simulink model "redundant_leg_final"  (R2024a)
settings: Solver=ode23tb  StartTime=0.0  StopTime=1  RelTol=1e-3
libraries: spsMosfetLib x6, spsIdealSwitchLib x4, spsCurrentMeasurementLib x3, spsDCVoltageSourceLib x1, spsSeriesRLCBranchLib x1, spsTriangleGeneratorLib x1, spsVoltageMeasurementLib x1, sps_lib x1
settings Model: Creator=student  LastModifiedBy=Rupa
settings SolverCC: ZeroCrossControl=DisableAll
settings RTWCC: GPUComputeCapability=3.5

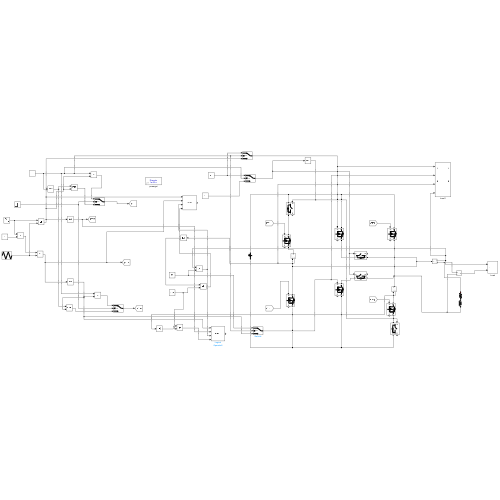
[thumbnail: Simulink's stored preview of the top-level diagram]
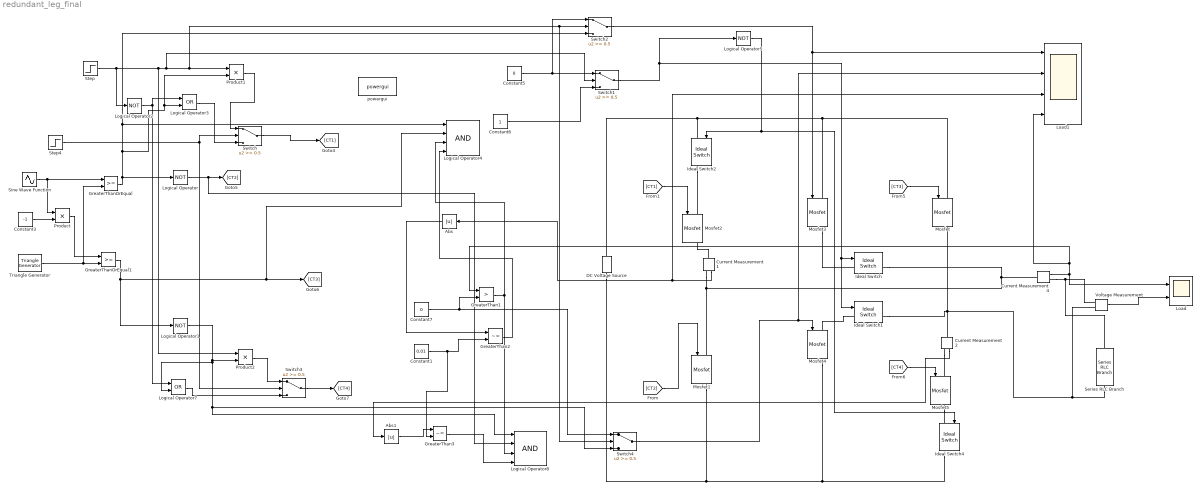
== system redundant_leg_final ==
  Abs : Abs  SaturateOnIntegerOverflow=off
  Abs1 : Abs  SaturateOnIntegerOverflow=off
  Constant1 : Constant  Value=0.01
  Constant3 : Constant  Value=-1
  Constant5 : Constant  Value=0
  Constant6 : Constant
  Constant7 : Constant  Value=0
  Current Measurement1 : spsCurrentMeasurementLib/Current Measurement  PhasorSimulation=off  OutputType=Complex  PSBequivalent=0
  Current Measurement2 : spsCurrentMeasurementLib/Current Measurement  PhasorSimulation=off  OutputType=Complex  PSBequivalent=0
  Current Measurement4 : spsCurrentMeasurementLib/Current Measurement  PhasorSimulation=off  OutputType=Complex  PSBequivalent=0
  DC Voltage Source : spsDCVoltageSourceLib/DC Voltage Source  Amplitude=200  Measurements=None
  GreaterThan1 : RelationalOperator  Operator=>  OutDataTypeStr=boolean  RndMeth=Simplest  InputSameDT=off
  GreaterThan2 : RelationalOperator  Operator=~=  OutDataTypeStr=boolean  RndMeth=Simplest  InputSameDT=off
  GreaterThan3 : RelationalOperator  Operator=~=  OutDataTypeStr=boolean  RndMeth=Simplest  InputSameDT=off
  GreaterThanOrEqual : RelationalOperator  OutDataTypeStr=boolean  RndMeth=Simplest  InputSameDT=off
  GreaterThanOrEqual1 : RelationalOperator  OutDataTypeStr=boolean  RndMeth=Simplest  InputSameDT=off
  Ideal Switch{,1..2,4} (4 alike) : spsIdealSwitchLib/Ideal Switch  Ron=0.001  Lon=0  IC=0  Rs=1e5  Cs=inf  Measurements=on
  Load : Scope  NumInputPorts=2
  Load1 : Scope  NumInputPorts=4
  Logical Operator{,1..2,5} (4 alike) : Logic  Operator=NOT  AllPortsSameDT=off  OutDataTypeStr=boolean
  Logical Operator3 : Logic  Operator=OR  AllPortsSameDT=off  OutDataTypeStr=boolean
  Logical Operator4 : Logic  Inputs=4  AllPortsSameDT=off  OutDataTypeStr=boolean
  Logical Operator7 : Logic  Operator=OR  AllPortsSameDT=off  OutDataTypeStr=boolean
  Logical Operator8 : Logic  Inputs=4  AllPortsSameDT=off  OutDataTypeStr=boolean
  Mosfet{,1..5} (6 alike) : spsMosfetLib/Mosfet  Ron=0.1  Lon=0  Rd=0.01  Vfd=0  IC=0  Rs=1e5  Cs=inf  Measurements=on
  Product : Product
  Product1 : Product
  Product2 : Product
  Series RLC Branch : spsSeriesRLCBranchLib/Series RLC Branch  LConnTagsString=__new0  RConnTagsString=__new0  BranchType=RL  Resistance=4  Inductance=5.3e-3  SetiL0=off  InitialCurrent=0  Capacitance=1e-6  Setx0=off  InitialVoltage=0  Measurements=None
  Sine Wave Function : Sin  Amplitude=0.9  Frequency=314.15  SampleTime=0
  Step : Step  Time=0.5  Before=1  After=0  SampleTime=0
  Step4 : Step  Time=.1  SampleTime=0
  Switch{,1..4} (5 alike) : Switch  Threshold=0.5  SaturateOnIntegerOverflow=off  InputSameDT=off
  Triangle Generator : spsTriangleGeneratorLib/Triangle Generator  Freq=3000  Phase=90  Ts=0
  Voltage Measurement : spsVoltageMeasurementLib/Voltage Measurement  PhasorSimulation=off  OutputType=Complex  PSBequivalent=0
  powergui : sps_lib/powergui  Priority=1  SimulationMode=Discrete  SampleTime=10e-6  frequency=60  Iterations=50  frequencyindice=0  Pbase=100e6  ErrMax=1e-4  UnitsV=kV  UnitsW=MW  buscounter=0  FunctionMessages=off  echomessages=off  EnableUseOfTLC=off  CurrentSourceSwitches=off  DisableSnubberDevices=off  DisableRonSwitches=off  DisableVfSwitches=off  DisplayEquations=off  AutomaticDiscreteSolvers=off  SolverType=Tustin/Backward Euler (TBE)  Interpol=off  ExternalGateDelay=off  methode=off  Ts=100  x0status=blocks  SPID=on  SwTol=0  HookPort=off  NonlinearTolerance=1e-4  nMaxIteration=100  ContinueOnMaxIteration=off  RestoreLinks=warning  ResistiveCurrentMeasurement=off  Frange=[0:2:500]  Ylog=off  Xlog=on  ShowGrid=off  save=off  variable=ZData  structure=0  ZoomFFT=off  StartTime=0.0  cycles=1  DisplayStyle=1  fundamental=60  FreqAxis=off  MaxFrequency=1000  frequencyindicesteady=1  RmsSteady=1  display=off
  wires:
  GreaterThanOrEqual/1 -> Logical Operator/1, Switch2/3, Logical Operator4/1, Logical Operator3/2, Product1/2
  Sine Wave Function/1 -> GreaterThanOrEqual/1, Product/1
  Triangle Generator/1 -> GreaterThanOrEqual1/2, GreaterThanOrEqual/2
  Constant3/1 -> Product/2
  Product/1 -> GreaterThanOrEqual1/1
  Step/1 -> Product2/1, Switch1/2, Switch4/2, Switch2/2, Product1/1, Logical Operator2/1
  Product1/1 -> Switch/1
  Logical Operator2/1 -> Logical Operator7/1, Logical Operator3/1
  Logical Operator3/1 -> Switch/3
  GreaterThanOrEqual1/1 -> Logical Operator1/1, Logical Operator4/2, [CT3]
  Step4/1 -> Switch3/2, Switch/2
  Logical Operator/1 -> Logical Operator8/2, [CT2]
  Logical Operator1/1 -> Logical Operator8/1, Switch4/3, Logical Operator7/2, Product2/2
  Current Measurement4/1 -> Load1/4, GreaterThan1/1, Load/1
  Constant7/1 -> Switch4/1, GreaterThan1/2
  GreaterThan1/1 -> Logical Operator8/3, Logical Operator4/3
  Switch/1 -> [CT1]
  Abs/1 -> GreaterThan2/1
  Constant1/1 -> GreaterThan3/2, GreaterThan2/2
  Voltage Measurement/1 -> Load/2
  [CT2] -> Mosfet1/1
  [CT4] -> Mosfet5/1
  Current Measurement1/1 -> Load1/3, Abs/1
  [CT3] -> Mosfet/1
  Constant5/1 -> Switch2/1, Switch1/1
  Constant6/1 -> Switch1/3
  Switch1/1 -> Ideal Switch1/1, Ideal Switch/1, Logical Operator5/1
  GreaterThan2/1 -> Logical Operator4/4
  [CT1] -> Mosfet2/1
  Switch2/1 -> Load1/1, Mosfet3/1
  Logical Operator5/1 -> Ideal Switch2/1, Ideal Switch4/1
  Logical Operator7/1 -> Switch3/3
  Product2/1 -> Switch3/1
  Switch3/1 -> [CT4]
  Abs1/1 -> GreaterThan3/1
  Current Measurement2/1 -> Abs1/1
  GreaterThan3/1 -> Logical Operator8/4
  Switch4/1 -> Load1/2, Mosfet4/1
  connections:
  Current Measurement4/RConn1 -- Series RLC Branch/LConn1 -- Voltage Measurement/LConn1
  Ideal Switch4/RConn1 -- Mosfet1/RConn1 -- DC Voltage Source/LConn1 -- Mosfet4/RConn1
  Mosfet3/LConn1 -- Mosfet/LConn1 -- DC Voltage Source/RConn1 -- Ideal Switch2/LConn1
  Ideal Switch1/RConn1 -- Current Measurement2/LConn1 -- Voltage Measurement/LConn2 -- Series RLC Branch/RConn1 -- Mosfet/RConn1
  Mosfet5/RConn1 -- Ideal Switch4/LConn1
  Ideal Switch2/RConn1 -- Mosfet2/LConn1
  Mosfet3/RConn1 -- Ideal Switch/LConn1
  Mosfet2/RConn1 -- Current Measurement1/LConn1
  Current Measurement1/RConn1 -- Ideal Switch/RConn1 -- Current Measurement4/LConn1 -- Mosfet1/LConn1
  Ideal Switch1/LConn1 -- Mosfet4/LConn1
  Current Measurement2/RConn1 -- Mosfet5/LConn1
